simulink model "VFD"  (R2022b)
settings: Solver=VariableStepAuto  StartTime=0.0  StopTime=10.0  RelTol=1e-3
libraries: spsMosfetLib x6, simulink x2, spsAsynchronousMachinepuUnitsLib x1, spsDCVoltageSourceLib x1, sps_lib x1
settings Model: Creator=User  LastModifiedBy=User

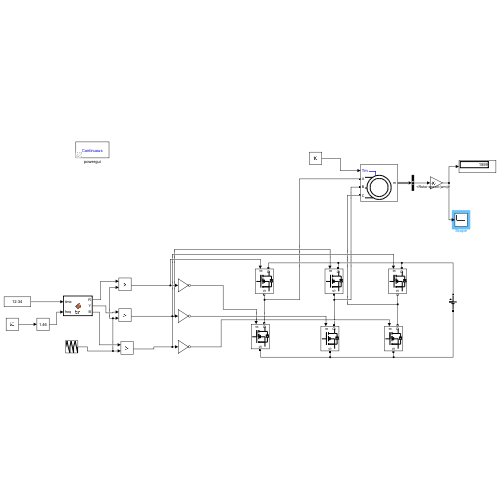
[thumbnail: Simulink's stored preview of the top-level diagram]
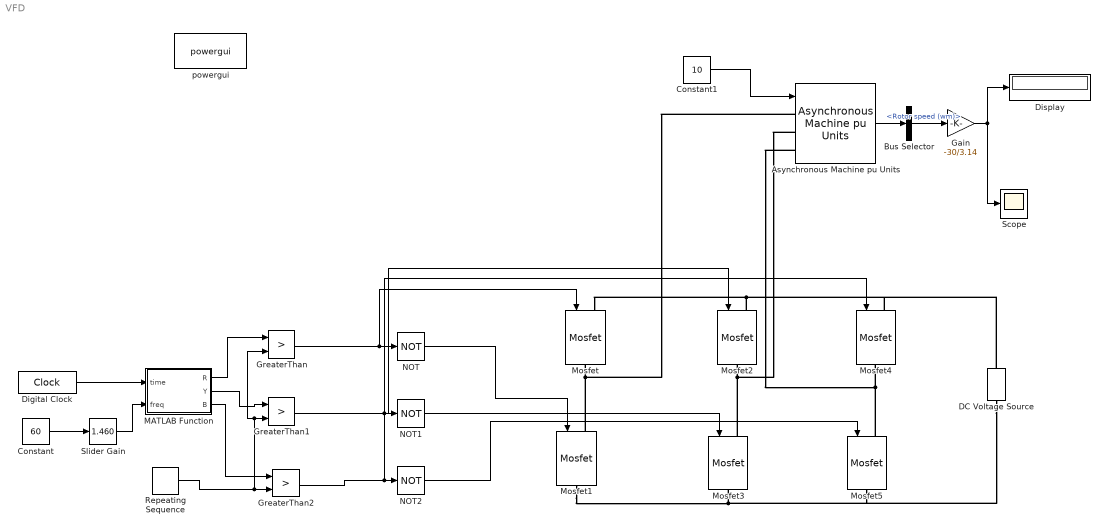
== system VFD ==
  Asynchronous Machine pu Units : spsAsynchronousMachinepuUnitsLib/Asynchronous Machine pu Units  RotorType=Squirrel-cage  PresetModel=No  MechanicalLoad=Torque Tm  ShowDetailedParameters=on  ReferenceFrame=Rotor  Units=pu  MeasurementBus=off  NominalParameters=[3730 460 60]  VoltageRatio=1  Stator=[0.01965 0.0397]  Rotor=[0.01909 0.0397]  Cage1=[0.01909 0.0397]  Cage2=[0.01909 0.0397]  Lm=1.354  Mechanical=[0.09526 0.05479 2]  PolePairs=2  InitialConditions="[ 1,0   0,0,0   0,0,0 ]"  SimulateSaturation=off  Saturation="[0.212,0.4201,0.8125,1.0979,1.4799,2.2457,3.2586,4.5763,6.4763 ;   0.5,0.7,0.9,1,1.1,1.2 ,1.3,1.4,1.5]"  LoadFlowParameters=0  TsPowergui=0  TsBlock=-1  IterativeModel=Trapezoidal non iterative  IterativeDiscreteModel=Trapezoidal non iterative  Pmec=0
      settings: LibrarySourceBlock=|
      | sps_lib/Electrical Machines/Asynchronous Machine
      | pu Units
  Bus Selector : BusSelector  OutputSignals=Mechanical.Rotor speed (wm)
  Constant : Constant  Value=60
  Constant1 : Constant  Value=10
  DC Voltage Source : spsDCVoltageSourceLib/DC Voltage Source  Amplitude=500  Measurements=None
  Digital Clock : DigitalClock
  Display : Display
  Gain : Gain  Gain=-30/3.14
  GreaterThan : RelationalOperator  Operator=>  OutDataTypeStr=boolean  RndMeth=Simplest  InputSameDT=off
  GreaterThan1 : RelationalOperator  Operator=>  OutDataTypeStr=boolean  RndMeth=Simplest  InputSameDT=off
  GreaterThan2 : RelationalOperator  Operator=>  OutDataTypeStr=boolean  RndMeth=Simplest  InputSameDT=off
  MATLAB Function : MATLAB Function  TreatAsAtomicUnit=on
  Mosfet{,1..5} (6 alike) : spsMosfetLib/Mosfet  Ron=0.1  Lon=0  Rd=0.01  Vfd=0  IC=0  Rs=1e5  Cs=inf  Measurements=off
  NOT : Logic  Operator=NOT  IconShape=distinctive  AllPortsSameDT=off  OutDataTypeStr=boolean
  NOT1 : Logic  Operator=NOT  IconShape=distinctive  AllPortsSameDT=off  OutDataTypeStr=boolean
  NOT2 : Logic  Operator=NOT  IconShape=distinctive  AllPortsSameDT=off  OutDataTypeStr=boolean
  Repeating Sequence : simulink/Sources/Repeating Sequence  rep_seq_t=[0.25 .5 .75 1]/5000  rep_seq_y=[0 1 0 -1]
  Scope : Scope
  Slider Gain : simulink/Math Operations/Slider Gain  gain=1.460  low=0  high=2
  powergui : sps_lib/powergui  Priority=1  SimulationMode=Continuous  SampleTime=50e-6  frequency=60  Iterations=50  frequencyindice=60  Pbase=100e6  ErrMax=1e-4  UnitsV=kV  UnitsW=MW  buscounter=0  FunctionMessages=off  echomessages=off  EnableUseOfTLC=off  CurrentSourceSwitches=off  DisableSnubberDevices=off  DisableRonSwitches=off  DisableVfSwitches=off  DisplayEquations=off  AutomaticDiscreteSolvers=off  SolverType=Tustin/Backward Euler (TBE)  Interpol=off  ExternalGateDelay=off  methode=off  Ts=100  x0status=blocks  SPID=on  SwTol=0  HookPort=off  NonlinearTolerance=1e-4  nMaxIteration=100  ContinueOnMaxIteration=off  RestoreLinks=warning  ResistiveCurrentMeasurement=off  Frange=[0:2:500]  Ylog=off  Xlog=on  ShowGrid=off  save=off  variable=ZData  structure=0  ZoomFFT=off  StartTime=0.0  cycles=1  DisplayStyle=1  fundamental=60  FreqAxis=off  MaxFrequency=1000  frequencyindicesteady=1  RmsSteady=1  display=off
  wires:
  Digital Clock/1 -> MATLAB Function/1(time)
  Constant/1 -> Slider Gain/1
  Slider Gain/1 -> MATLAB Function/2(freq)
  MATLAB Function/1(R) -> GreaterThan/1
  MATLAB Function/2(Y) -> GreaterThan1/1
  MATLAB Function/3(B) -> GreaterThan2/1
  Repeating Sequence/1 -> GreaterThan/2, GreaterThan1/2, GreaterThan2/2
  GreaterThan2/1 -> Mosfet4/1, NOT2/1
  GreaterThan1/1 -> Mosfet2/1, NOT1/1
  GreaterThan/1 -> Mosfet/1, NOT/1
  NOT/1 -> Mosfet1/1
  NOT1/1 -> Mosfet3/1
  NOT2/1 -> Mosfet5/1
  Constant1/1 -> Asynchronous Machine pu Units/1
  Gain/1 -> Display/1, Scope/1
  Asynchronous Machine pu Units/1 -> Bus Selector/1
  Bus Selector/1 -> Gain/1  "<Rotor speed (wm)>"
  connections:
  Mosfet3/LConn1 -- Asynchronous Machine pu Units/LConn2 -- Mosfet2/RConn1
  Mosfet5/LConn1 -- Asynchronous Machine pu Units/LConn3 -- Mosfet4/RConn1
  Mosfet2/LConn1 -- DC Voltage Source/RConn1 -- Mosfet4/LConn1 -- Mosfet/LConn1
  Mosfet1/LConn1 -- Asynchronous Machine pu Units/LConn1 -- Mosfet/RConn1
  Mosfet1/RConn1 -- DC Voltage Source/LConn1 -- Mosfet5/RConn1 -- Mosfet3/RConn1

== matlab function VFD/MATLAB Function ==
  data: time input; R output; freq input; Y output; B output
function [R ,Y,B]= fcn(time,freq)
omega =2*pi*freq;
R =(freq/60)*(omega*time);
Y =(freq/60)*(omega*time+120*pi/180);
B =(freq/60)*(omega*time+240*pi/180);
